simulink model "CIFB"  (R2022b)
settings: Solver=FixedStepDiscrete  StartTime=0.0  StopTime=0.01  RelTol=1e-3
libraries: dspsrcs4 x1
settings Model: Creator=ASAA  LastModifiedBy=ASAA

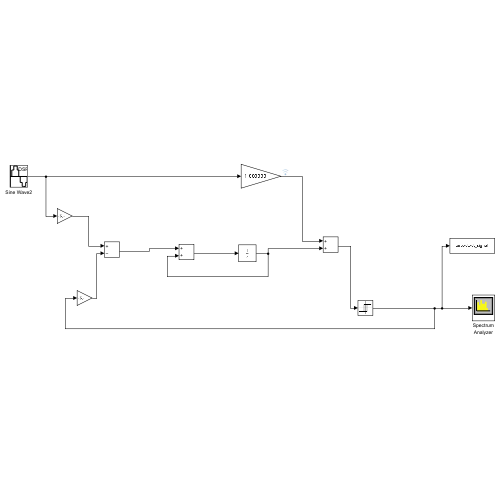
[thumbnail: Simulink's stored preview of the top-level diagram]
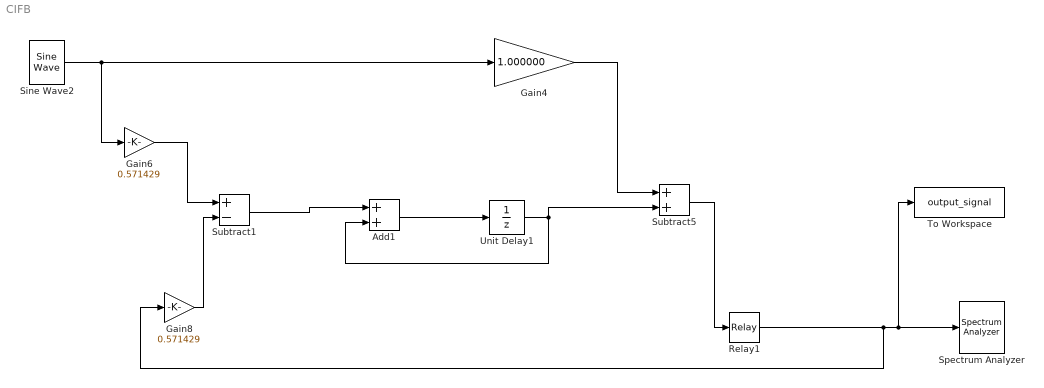
== system CIFB ==
  Add1 : Sum
  Gain4 : Gain  Gain=1.000000
  Gain6 : Gain  Gain=0.571429
  Gain8 : Gain  Gain=0.571429
  Relay1 : Relay  OffOutputValue=-1
  Sine Wave2 : dspsrcs4/Sine Wave  Amplitude=0.63  Frequency=100e3  Phase=0  SampleMode=Discrete  OutComplex=Real  CompMethod=Trigonometric fcn  TableSize=Speed  SampleTime=1e-8  SamplesPerFrame=1  ResetState=Restart at time zero  OutputFrames=off  dataType=double  wordLen=16  udDataType=sfix(16)  fracBitsMode=Best precision  numFracBits=15  OutDataTypeStr=double  LastOutDataTypeStr=double
  Spectrum Analyzer : SpectrumAnalyzer
  Subtract1 : Sum  Inputs=+-
  Subtract5 : Sum
  To Workspace : ToWorkspace  VariableName=output_signal  SaveFormat=Timeseries  SampleTime=-1
  Unit Delay1 : UnitDelay  SampleTime=-1  HasFrameUpgradeWarning=on
  wires:
  Relay1/1 -> To Workspace/1, Spectrum Analyzer/1, Gain8/1
  Gain6/1 -> Subtract1/1
  Gain4/1 -> Subtract5/1
  Subtract5/1 -> Relay1/1
  Gain8/1 -> Subtract1/2
  Sine Wave2/1 -> Gain6/1, Gain4/1
  Add1/1 -> Unit Delay1/1
  Subtract1/1 -> Add1/1
  Unit Delay1/1 -> Subtract5/2, Add1/2
